simulink model "induction_motor_vf"  (R2021a)
settings: Solver=VariableStepAuto  StartTime=0.0  StopTime=5  RelTol=1e-3
libraries: spsAsynchronousMachineSIUnitsLib x1, spsDCVoltageSourceLib x1, eeAsmScalarControl x1, eePwmGeneratorTwoLevel x1, simulink x1, spsUniversalBridgeLib x1, spsVoltageMeasurementLib x1, spspowerguiLib x1
settings Model: Creator=Prakhar  LastModifiedBy=Prakhar

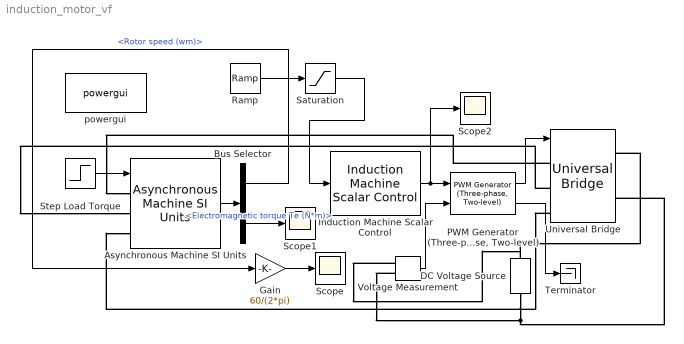
== system induction_motor_vf ==
  Asynchronous Machine SI Units : spsAsynchronousMachineSIUnitsLib/Asynchronous Machine SI Units  RotorType=Squirrel-cage  PresetModel=No  MechanicalLoad=Torque Tm  ShowDetailedParameters=on  ReferenceFrame=Rotor  Units=SI  MeasurementBus=off  NominalParameters=[5.5e3 400 50]  VoltageRatio=1  Stator=[0.5 0.00382]  Rotor=[0.3 0.002546]  Cage1=[0.4155 0.002066]  Cage2=[0.4168 0.0003495]  Lm=0.09549  Mechanical=[0.05 0.001 2]  PolePairs=2  InitialConditions=[1 0 0 0 0 0 0 0]  SimulateSaturation=off  Saturation=[14.03593122, 27.81365428, 53.79336849, 72.68890987, 97.98006896, 148.6815601, 215.7428561, 302.9841135, 428.7778367 ; 230, 322, 414, 460, 506, 552, 598, 644, 690]  LoadFlowParameters=1492000  TsPowergui=0  TsBlock=-1  IterativeModel=Trapezoidal non iterative  IterativeDiscreteModel=Trapezoidal non iterative  Pmec=1.492e+006
  Bus Selector : BusSelector  OutputSignals=Mechanical.Rotor speed (wm),Mechanical.Electromagnetic torque Te (N*m)
  DC Voltage Source : spsDCVoltageSourceLib/DC Voltage Source  Amplitude=700  Measurements=Voltage
  Gain : Gain  Gain=60/(2*pi)
  Induction Machine Scalar Control : eeAsmScalarControl/Induction Machine Scalar Control  fn=50  Vn=400  Vmin=10  Ts=-1
      settings: SourceProductBaseCode=PS
  "PWM Generator (Three-phase, Two-level)" : eePwmGeneratorTwoLevel/PWM Generator (Three-phase, Two-level)  PWMMode=Continuous PWM (CPWM)  CPWMMode=SPWM: sinusoidal PWM  DPWMMode=60 DPWM: 60 degree discontinuous PWM  fsw=5000  Ts=5e-6
      settings: SourceProductBaseCode=PS
  Ramp : simulink/Sources/Ramp  slope=30  start=0  InitialOutput=0
  Saturation : Saturate  UpperLimit=30  LowerLimit=0
  Scope : Scope
  Scope1 : Scope
  Scope2 : Scope
  Step Load Torque : Step  After=20  SampleTime=0
  Terminator : Terminator
  Universal Bridge : spsUniversalBridgeLib/Universal Bridge  Arms=3  SnubberResistance=1e5  SnubberCapacitance=inf  Device=IGBT / Diodes  Ron=1e-3  Lon=0  ForwardVoltages="[  0  0  ]"  ForwardVoltage=0  GTOparameters=[ 10e-6 , 20e-6 ]  IGBTparameters=[ 1e-6 , 2e-6 ]  Measurements=None  Measurements_2=None  converterType=Rectifier
  Voltage Measurement : spsVoltageMeasurementLib/Voltage Measurement  PhasorSimulation=off  OutputType=Complex  PSBequivalent=0
  powergui : spspowerguiLib/powergui  Priority=1  SimulationMode=Continuous  SampleTime=50e-6  frequency=60  Iterations=50  frequencyindice=50  Pbase=100e6  ErrMax=1e-4  UnitsV=kV  UnitsW=MW  buscounter=0  FunctionMessages=off  echomessages=off  EnableUseOfTLC=off  CurrentSourceSwitches=off  DisableSnubberDevices=off  DisableRonSwitches=off  DisableVfSwitches=off  DisplayEquations=off  AutomaticDiscreteSolvers=off  SolverType=Tustin/Backward Euler (TBE)  Interpol=off  ExternalGateDelay=off  methode=off  Ts=100  x0status=blocks  SPID=on  SwTol=0  HookPort=off  NonlinearTolerance=1e-4  nMaxIteration=100  ContinueOnMaxIteration=off  RestoreLinks=warning  ResistiveCurrentMeasurement=off  Frange=[0:2:500]  Ylog=off  Xlog=on  ShowGrid=off  save=off  variable=ZData  structure=0  ZoomFFT=off  StartTime=0.0  cycles=1  DisplayStyle=1  fundamental=60  FreqAxis=off  MaxFrequency=1000  frequencyindicesteady=1  RmsSteady=1  display=off
  wires:
  Step Load Torque/1 -> Asynchronous Machine SI Units/1
  Induction Machine Scalar Control/1 -> Scope2/1, "PWM Generator (Three-phase, Two-level)"/1
  "PWM Generator (Three-phase, Two-level)"/1 -> Universal Bridge/1
  Voltage Measurement/1 -> "PWM Generator (Three-phase, Two-level)"/2
  Asynchronous Machine SI Units/1 -> Bus Selector/1
  Bus Selector/1 -> Gain/1  "<Rotor speed (wm)>"
  Gain/1 -> Scope/1
  "PWM Generator (Three-phase, Two-level)"/2 -> Terminator/1
  Bus Selector/2 -> Scope1/1  "<Electromagnetic torque Te (N*m)>"
  Saturation/1 -> Induction Machine Scalar Control/1
  Ramp/1 -> Saturation/1
  connections:
  DC Voltage Source/RConn1 -- Voltage Measurement/LConn1 -- Universal Bridge/RConn1
  Universal Bridge/LConn1 -- Asynchronous Machine SI Units/LConn1
  Universal Bridge/LConn2 -- Asynchronous Machine SI Units/LConn2
  Universal Bridge/LConn3 -- Asynchronous Machine SI Units/LConn3
  DC Voltage Source/LConn1 -- Universal Bridge/RConn2 -- Voltage Measurement/LConn2
